simulink model "testrig_AirOilPiston_multibody"  (R2026b)
settings: Solver=daessc  StopTime=25  MaxStep=1e-2  AbsTol=1e-3
PreLoadFcn:
  | Spring = VDatabase.Spring.SUV_Landy_TA2PR_AirOilPiston_A1;
  | mass_sprung = 436.5;
  | load testrig_AirOilPiston_roughroad
undefined symbols (not defined in the file or in its folder): X, Y, Z
libraries: sm_lib x8, nesl_utility x3, fl_lib x2, Spring_AirOilPiston x1, testrig_AirOilPiston_lib x1
settings Model: Creator=Glenn  LastModifiedBy=smiller
settings SolverCC: AutoScaleAbsTol=off  MaxConsecutiveMinStep=5
settings DataIOCC: ReturnWorkspaceOutputs=off  SignalLoggingName=logsout_testrig_AirOilPiston
settings SimscapeCC: SimscapeLogLimitData=off  SimscapeLogName=simlog_testrig_AirOilPiston  SimscapeLogType=all  SimscapeUseEnergyAccounting=off
settings ExplorerConfigSet: InternalSimMechanicsExplorerSettings="<ExplorerConfiguration><canonicalview>default</canonicalview><AnimationSetting><BasePlaybackSpeed>1.0</BasePlaybackSpeed><PlaybackSpeedFactor>2.0</PlaybackSpeedFactor></AnimationSetting><TilePanel><TileInfo><Tiles Columns=\"1\" Count=\"1\" Rows=\"1\"><Column Weight=\"1\"/><Row Weight=\"1\"/><Tile Height=\"1\" Width=\"1\" X=\"0\" Y=\"0\"/></Tiles></TileInfo><SceneInfo><SceneViewer><BGColor><R>0.60000002384185791</R><G>0.60000002384185791</G><B>0.60000002384185791</B></BGColor><Camera><DoPerspective>off</DoPerspective><Position><X>0.840069872001566131</X><Y>-0.587067130109622304</Y><Z>0.736508931620452945</Z></Position><Center><X>0.0636729707701644276</X><Y>-0.0264759743902784582</Y><Z>0.448506487381626129</Z></Center><Up><X>-0.244728224943584149</X><Y>0.152949790100556315</Y><Z>0.957452065444614364</Z></Up><ViewLimDist>1</ViewLimDist><YLim>1.03004967622777266</YLim><XLim>0.912665097740277154</XLim></Camera></SceneViewer></SceneInfo></TilePanel><MechEditorPanel><Cameras/><GfxPanelCameraMap/><VideoCreator><PlaybackSpeedRatio>1.0</PlaybackSpeedRatio><FrameRate>30</FrameRate><VideoFormat>Motion JPEG AVI</VideoFormat><FrameSize>auto</FrameSize></VideoCreator></MechEditorPanel></ExplorerConfiguration>"

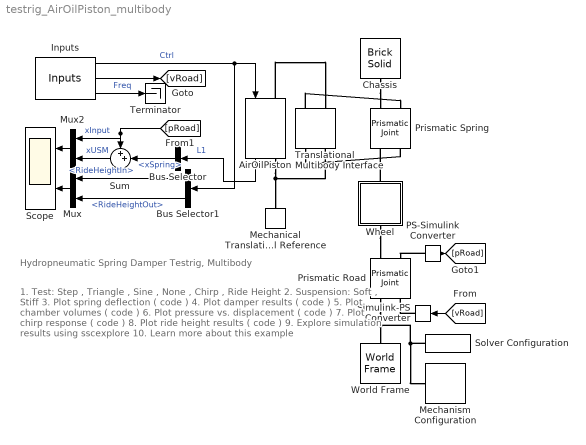
== system testrig_AirOilPiston_multibody ==
  note: 1. Test: Step , Triangle , Sine , None , Chirp , Ride Height
      | 2. Suspension: Soft , Stiff
      | 3. Plot spring deflection ( code )
      | 4. Plot damper results ( code )
      | 5. Plot chamber volumes ( code )
      | 6. Plot pressure vs. displacement ( code )
      | 7. Plot chirp response ( code )
      | 8. Plot ride height results ( code )
      | 9. Explore simulation results using sscexplore
      | 10. Learn more about this example
  note: Hydropneumatic Spring Damper Testrig, Multibody
  AirOilPiston : Spring_AirOilPiston/AirOilPiston  spr_hp_top=Spring.sTop.Value*0  spr_hp_bot=Spring.sBottom.Value*0  t_ambient=Spring.Spring.TAmbient.Value  gspr_gas_properties=Spring.Spring.GasProperties  strut_oil_properties=Spring.Strut.OilProperties  gas_chamber_soft_area=Spring.Spring.GasSoft.A.Value  gas_chamber_stiff_area=Spring.Spring.GasStiff.A.Value  gas_chamber_soft_deadvol=Spring.Spring.GasSoft.volDead.Value  gas_chamber_stiff_deadvol=Spring.Spring.GasStiff.volDead.Value  gspr_mass_soft=Spring.Spring.GasSoft.mPiston.Value  gspr_mass_stiff=Spring.Spring.GasStiff.mPiston.Value  gspr_damping_soft=Spring.Spring.GasSoft.b.Value  gspr_damping_stiff=Spring.Spring.GasStiff.b.Value  gas_chamber_soft_x0=Spring.Spring.GasSoft.xInit.Value  gas_chamber_stiff_x0=Spring.Spring.GasStiff.xInit.Value  gas_chamber_soft_p0=Spring.Spring.GasSoft.pInit.Value  gas_chamber_stiff_p0=Spring.Spring.GasStiff.pInit.Value  gspr_cwall_soft=Spring.Spring.GasSoft.CWall.Value  gspr_cwall_stiff=Spring.Spring.GasStiff.CWall.Value  oil_chamber_soft_area=Spring.Spring.OilSoft.A.Value  oil_chamber_stiff_area=Spring.Spring.OilStiff.A.Value  oil_chamber_soft_deadvol=Spring.Spring.OilSoft.volDead.Value  oil_chamber_stiff_deadvol=Spring.Spring.OilStiff.volDead.Value  oil_chamber_soft_x0=Spring.Spring.OilSoft.xInit.Value  oil_chamber_stiff_x0=Spring.Spring.OilStiff.xInit.Value  oil_chamber_soft_p0=Spring.Spring.OilSoft.pInit.Value  oil_chamber_stiff_p0=Spring.Spring.OilStiff.pInit.Value  gsprv_smax_soft=Spring.Spring.ValveSoft.xMaxOpen.Value  gsprv_smax_stiff=Spring.Spring.ValveStiff.xMaxOpen.Value  gsprv_delsmax_soft=Spring.Spring.ValveSoft.xCloseToOpen.Value  gsprv_delsmax_stiff=Spring.Spring.ValveStiff.xCloseToOpen.Value  gsprv_arealeak_soft=Spring.Spring.ValveSoft.areaLeak.Value  gsprv_arealeak_stiff=Spring.Spring.ValveStiff.areaLeak.Value  gsprv_areamax_soft=Spring.Spring.ValveSoft.aMax.Value  gsprv_areamax_stiff=Spring.Spring.ValveStiff.aMax.Value  gsprv_cd_soft=Spring.Spring.ValveSoft.Cd.Value  gsprv_cd_stiff=Spring.Spring.ValveStiff.Cd.Value  gsprv_smooth_soft=Spring.Spring.ValveSoft.smoothFactor.Value  gsprv_smooth_stiff=Spring.Spring.ValveStiff.smoothFactor.Value  gsprva_stroke_soft=Spring.Spring.ValveActuatorSoft.xStroke.Value  gsprva_stroke_stiff=Spring.Spring.ValveActuatorStiff.xStroke.Value  gsprva_ton_soft=Spring.Spring.ValveActuatorSoft.tOn.Value  gsprva_ton_stiff=Spring.Spring.ValveActuatorStiff.tOn.Value  gsprva_toff_soft=Spring.Spring.ValveActuatorSoft.tOff.Value  gsprva_toff_stiff=Spring.Spring.ValveActuatorStiff.tOff.Value  strut_deadvol=Spring.Strut.volDead.Value  strut_area=Spring.Strut.A.Value  strut_x0=Spring.Strut.xInit.Value  strut_frc_colfrc=Spring.Strut.Friction.fCoulomb.Value  strut_frc_brkfrc=Spring.Strut.Friction.fBreakaway.Value  strut_frc_brkvel=Spring.Strut.Friction.vBreakaway.Value  strut_frc_visccoeff=Spring.Strut.Friction.mu.Value  strut_p0=Spring.Strut.pInit.Value  bs_lim_upper=Spring.Endstop.xMax.Value  bs_lim_lower=Spring.Endstop.xMin.Value  bs_k_upper=Spring.Endstop.KxMax.Value  bs_k_lower=Spring.Endstop.KxMin.Value  bs_b_upper=Spring.Endstop.dxMax.Value  bs_b_lower=Spring.Endstop.dxMin.Value  bs_region=Spring.Endstop.xTransition.Value  p_diff_TLU_constant=Spring.Damper.Orifice.pDiff.Value  vol_flow_TLU_constant=Spring.Damper.Orifice.q.Value  dpr_restrarea_comp=Spring.Damper.RestrictionComp.A.Value  dpr_restrarea_reb=Spring.Damper.RestrictionReb.A.Value  dpr_cd_comp=Spring.Damper.RestrictionComp.Cd.Value  dpr_cd_reb=Spring.Damper.RestrictionReb.Cd.Value  dpr_prv_psetdiff_comp=Spring.Damper.PRVComp.pDiff.Value  dpr_prv_psetdiff_reb=Spring.Damper.PRVReb.pDiff.Value  dpr_prv_prange_comp=Spring.Damper.PRVComp.pRange.Value  dpr_prv_prange_reb=Spring.Damper.PRVReb.pRange.Value  dpr_prv_areamax_comp=Spring.Damper.PRVComp.A.Value  dpr_prv_areamax_reb=Spring.Damper.PRVReb.A.Value  dpr_prv_cd_comp=Spring.Damper.PRVComp.Cd.Value  dpr_prv_cd_reb=Spring.Damper.PRVReb.Cd.Value  dpr_cvdvalve_cmpos=Spring.CVDValve.Orifice.x.Value  dpr_cvdvalve_orifice_area=Spring.CVDValve.Orifice.A.Value  dpr_cvdvalve_orifice_pdiff=Spring.CVDValve.Orifice.pDiff.Value  dpr_cvdvalve_pcv_areamax=Spring.CVDValve.PCValve.AMax.Value  dpr_cvdvalve_pcv_prange=Spring.CVDValve.PCValve.pRange.Value  dpr_cvdvalve_arealeak=Spring.CVDValve.PCValve.ALeak.Value  dpr_cvdvalve_cd=Spring.CVDValve.PCValve.Cd.Value  dpr_cvdvalve_act_ts=Spring.CVDValve.tFilt.Value  rh_srcpressure=Spring.RideHeight.pSource.Value  rh_fcv_cmpos_inlet=Spring.RideHeight.OrificeInlet.x.Value  rh_fcv_cmpos_outlet=Spring.RideHeight.OrificeOutlet.x.Value  rh_fcv_orificearea_inlet=Spring.RideHeight.OrificeInlet.A.Value  rh_fcv_orificearea_outlet=Spring.RideHeight.OrificeOutlet.A.Value  rh_fcv_orificepdiff_inlet=Spring.RideHeight.OrificeInlet.pDiff.Value  rh_fcv_orificepdiff_outlet=Spring.RideHeight.OrificeOutlet.pDiff.Value  rh_fcv_pcprange_inlet=Spring.RideHeight.PCValveInlet.pRange.Value  rh_fcv_pcprange_outlet=Spring.RideHeight.PCValveOutlet.pRange.Value  rh_fcv_pcamax_inlet=Spring.RideHeight.PCValveInlet.AMax.Value  rh_fcv_pcamax_outlet=Spring.RideHeight.PCValveOutlet.AMax.Value  rh_fcv_arealeak_inlet=Spring.RideHeight.PCValveInlet.ALeak.Value  rh_fcv_arealeak_outlet=Spring.RideHeight.PCValveOutlet.ALeak.Value  rh_fcv_cd_inlet=Spring.RideHeight.PCValveInlet.Cd.Value  rh_fcv_cd_outlet=Spring.RideHeight.PCValveOutlet.Cd.Value  rh_fcv_smooth_inlet=Spring.RideHeight.PCValveInlet.smoothFactor.Value  rh_fcv_smooth_outlet=Spring.RideHeight.PCValveOutlet.smoothFactor.Value  rh_fcv_tfilt_inlet=Spring.RideHeight.PCValveInlet.tFilt.Value  rh_fcv_tfilt_outlet=Spring.RideHeight.PCValveOutlet.tFilt.Value
  Bus Selector : BusSelector  OutputSignals=xSpring
  Bus Selector1 : BusSelector  OutputSignals=RideHeightIn,RideHeightOut
  Chassis : sm_lib/Body Elements/Brick Solid  BrickDimensions=[1 1 0.5]  BrickDimensionsUnits=m  ExportEntireGeometry=off  InertiaType=CalculateFromGeometry  BasedOnType=Mass  Density=1000  DensityUnits=kg/m^3  Mass=mass_sprung  MassUnits=kg  CenterOfMass=[0 0 0]  CenterOfMassUnits=m  MomentsOfInertia=[1 1 1]  MomentsOfInertiaUnits=kg*m^2  ProductsOfInertia=[0 0 0]  ProductsOfInertiaUnits=kg*m^2  GraphicType=FromGeometry  MarkerShape=Sphere  MarkerSize=10  GraphicVisPropType=SimpleVisualProperties  GraphicDiffuseColor=[0.1255 0.4706 0]  GraphicOpacity=1  GraphicSpecularColor=[0.5 0.5 0.5 1.0]  GraphicAmbientColor=[0.15 0.15 0.15 1.0]  GraphicEmissiveColor=[0.0 0.0 0.0 1.0]  GraphicShininess=75  DoExposeReferenceFrame=on  SerializedFrames=<Frames/>
  Inputs : testrig_AirOilPiston_lib/Inputs  popup_suspension_stiffness=Soft  popup_rh_test_seq=None  cvd_value=1  popup_roadpz_test_type=Step  pAmp=0.05  tPer=4  nCyc=50  nCycSet=1  chirpFreqFinish=5  chirpFreqStart=0.5  chirpTimeFinish=20  chirpTimeStart=5  spdkmh=10  roughTimeStart=5
      settings: AttributesFormatString=|
      | Road Height: %<popup_roadpz_test_type>
      | Suspension: %<popup_suspension_stiffness>
      | Ride Height: %<popup_rh_test_seq>
  Mechanical Translational Reference : fl_lib/Mechanical/Translational Elements/Mechanical Translational Reference
  Mechanism Configuration : sm_lib/Utilities/Mechanism Configuration  UniformGravity=Constant  GravityVector=[0 0 -9.80665]  GravityVectorUnits=m/s^2  LinearizationDelta=0.001  JointModeTransitionNonlinearIterations=2
  Mux : Mux  Inputs=2
  Mux2 : Mux  Inputs=2
  PS-Simulink Converter : nesl_utility/PS-Simulink Converter  PhysicalDomain=network_engine_domain  SubClassName=ps_output  LeftPortType=input  RightPortType=output  PseudoPeriodic=off  Frequencies=[]  VectorFormat=inherit  Unit=inherit  AffineConversion=off
  Prismatic Road : sm_lib/Joints/Prismatic Joint  JointMode=Normal  CompositeWrenchDir=FollowerOnBase  CompositeWrenchFrame=BaseFrame  SenseConstraintForce=off  SenseConstraintTorque=off  SenseTotalForce=off  SenseTotalTorque=off  PositionTargetSpecify=off  PositionTargetPriority=High  PositionTargetValue=0  PositionTargetValueUnits=m  VelocityTargetSpecify=off  VelocityTargetPriority=High  VelocityTargetValue=0  VelocityTargetValueUnits=m/s  EquilibriumPosition=0  EquilibriumPositionUnits=m  SpringStiffness=0  SpringStiffnessUnits=N/m  DampingCoefficient=0  DampingCoefficientUnits=N/(m/s)  LowerLimitSpecify=off  LowerLimitBound=-1  LowerLimitBoundUnits=m  LowerLimitStiffness=1e6  LowerLimitStiffnessUnits=N/m  LowerLimitDamping=1e3  LowerLimitDampingUnits=N/(m/s)  LowerLimitTransitionRegionWidth=1e-4  LowerLimitTransitionRegionWidthUnits=m  UpperLimitSpecify=off  UpperLimitBound=1  UpperLimitBoundUnits=m  UpperLimitStiffness=1e6  UpperLimitStiffnessUnits=N/m  UpperLimitDamping=1e3  UpperLimitDampingUnits=N/(m/s)  UpperLimitTransitionRegionWidth=1e-4  UpperLimitTransitionRegionWidthUnits=m  TorqueActuationMode=ComputedTorque  MotionActuationMode=InputMotion  SensePosition=on  SenseVelocity=off  SenseAcceleration=off  SenseTorqueForce=off  SenseLowerLimitTorqueForce=off  SenseUpperLimitTorqueForce=off
  Prismatic Spring : sm_lib/Joints/Prismatic Joint  JointMode=Normal  CompositeWrenchDir=FollowerOnBase  CompositeWrenchFrame=BaseFrame  SenseConstraintForce=off  SenseConstraintTorque=off  SenseTotalForce=off  SenseTotalTorque=off  PositionTargetSpecify=off  PositionTargetPriority=High  PositionTargetValue=0  PositionTargetValueUnits=m  VelocityTargetSpecify=off  VelocityTargetPriority=High  VelocityTargetValue=0  VelocityTargetValueUnits=m/s  EquilibriumPosition=0  EquilibriumPositionUnits=m  SpringStiffness=0  SpringStiffnessUnits=N/m  DampingCoefficient=0  DampingCoefficientUnits=N/(m/s)  LowerLimitSpecify=off  LowerLimitBound=-1  LowerLimitBoundUnits=m  LowerLimitStiffness=1e6  LowerLimitStiffnessUnits=N/m  LowerLimitDamping=1e3  LowerLimitDampingUnits=N/(m/s)  LowerLimitTransitionRegionWidth=1e-4  LowerLimitTransitionRegionWidthUnits=m  UpperLimitSpecify=off  UpperLimitBound=1  UpperLimitBoundUnits=m  UpperLimitStiffness=1e6  UpperLimitStiffnessUnits=N/m  UpperLimitDamping=1e3  UpperLimitDampingUnits=N/(m/s)  UpperLimitTransitionRegionWidth=1e-4  UpperLimitTransitionRegionWidthUnits=m  TorqueActuationMode=InputTorque  MotionActuationMode=ComputedMotion  SensePosition=off  SenseVelocity=on  SenseAcceleration=off  SenseTorqueForce=off  SenseLowerLimitTorqueForce=off  SenseUpperLimitTorqueForce=off
  Scope : Scope  NumInputPorts=2
      settings: ActiveDisplayYMinimum=-0.12106  ActiveDisplayYMaximum=0.26576
  Simulink-PS Converter : nesl_utility/Simulink-PS Converter  PhysicalDomain=network_engine_domain  SubClassName=ps_input  LeftPortType=input  RightPortType=output  PseudoPeriodic=off  Frequencies=[]  NoiseDistribution=none  NoiseParameters=[]  Unit=m  AffineConversion=off  FilteringAndDerivatives=filter  SimscapeFilterOrder=2  InputFilterTimeConstant=0.001  UdotUserProvided=0
  Solver Configuration : nesl_utility/Solver Configuration  PhysicalDomain=network_engine_domain  SubClassName=solver  LeftPortType=input  RightPortType=generic  Tones=[]  Harmonics=[]  SimulateNoise=off  Profile=off  UseLocalSampling=off  EnableSwitchedLinearOptims=on  FrequencyDomain=off  UseCCode=off  RelTol=0.001  AbsTol=0.001  MinStep=1e-09  ToWorkspace=off  RevertToSquareIcSolve=off  NumHomotopyIterations=100  PhasorMode=off  PhasorModeNumHarmonics=1  ConsistencySolver=NEWTON_FTOL  CanonicalOrdering=UNORDERED  OptimizeIntermediates=UNOPTIMIZED  MulticoreSolverChoice=BACKWARD_EULER  IndexReductionMethod=DerivativeReplacement  DoDC=off  ResidualTolerance=1e-09  ConsistencyTolSource=GLOBAL  ConsistencyAbsTol=0.001  ConsistencyRelTol=0.001  ConsistencyTolFactor=0.001  UseLocalSolver=off  LocalSolverChoice=NE_BACKWARD_EULER_ADVANCER  ResolveIndetEquations=on  FunctionEvalNumThread=1  LocalSolverSampleTime=0.001  DoFixedCost=off  MaxNonlinIter=3  MaxModeIter=2  ComputeImpulses=off  ImpulseIterations=2  LinearAlgebra=auto  LinearAlgebraNumThread=0  EquationFormulation=NE_TIME_EF  DelaysMemoryBudget=1024  AutomaticFiltering=on  FilteringTimeConstant=0.001  PartitionStorageMethod=AS_NEEDED  PartitionMemoryBudget=1024  PartitionMethod=BALANCED  MultibodyUseLocalSolver=off  MultibodyLocalSolverChoice=ODE1  MultibodyLocalSolverSampleTime=0.001
  Sum : Sum  Inputs=++|
  Terminator : Terminator
  Translational Multibody Interface : fl_lib/Mechanical/Multibody Interfaces/Translational Multibody Interface
  Wheel : Subsystem
  World Frame : sm_lib/Frames and Transforms/World Frame
  wires:
  AirOilPiston/1 -> Bus Selector/1  "L1"
  Sum/1 -> Mux2/2  "xUSM"
  Mux/1 -> Scope/2
  Bus Selector1/1 -> Mux/1  "<RideHeightIn>"
  Bus Selector1/2 -> Mux/2  "<RideHeightOut>"
  Inputs/1 -> Bus Selector1/1, AirOilPiston/1  "Ctrl"
  Mux2/1 -> Scope/1
  PS-Simulink Converter/1 -> [pRoad]
  [vRoad] -> Simulink-PS Converter/1
  [pRoad] -> Mux2/1, Sum/1  "xInput"
  Inputs/2 -> [vRoad]
  Bus Selector/1 -> Sum/2  "<xSpring>"
  Inputs/3 -> Terminator/1  "Freq"
  connections:
  AirOilPiston/RConn1 -- Translational Multibody Interface/LConn2 -- Mechanical Translational Reference/LConn1
  AirOilPiston/LConn1 -- Translational Multibody Interface/RConn2
  Translational Multibody Interface/LConn1 -- Prismatic Spring/LConn2
  Translational Multibody Interface/RConn1 -- Prismatic Spring/RConn2
  Chassis/RConn1 -- Prismatic Spring/RConn1
  Prismatic Road/LConn1 -- Mechanism Configuration/RConn1 -- Solver Configuration/RConn1 -- World Frame/RConn1
  Simulink-PS Converter/RConn1 -- Prismatic Road/LConn2
  PS-Simulink Converter/LConn1 -- Prismatic Road/RConn2
  Wheel/LConn1 -- Prismatic Spring/LConn1
  Wheel/RConn1 -- Prismatic Road/RConn1

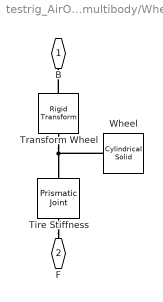
== system testrig_AirOilPiston_multibody/Wheel ==
  Tire Stiffness : sm_lib/Joints/Prismatic Joint  JointMode=Normal  CompositeWrenchDir=FollowerOnBase  CompositeWrenchFrame=BaseFrame  SenseConstraintForce=off  SenseConstraintTorque=off  SenseTotalForce=off  SenseTotalTorque=off  PositionTargetSpecify=off  PositionTargetPriority=High  PositionTargetValue=0  PositionTargetValueUnits=m  VelocityTargetSpecify=off  VelocityTargetPriority=High  VelocityTargetValue=0  VelocityTargetValueUnits=m/s  EquilibriumPosition=0  EquilibriumPositionUnits=m  SpringStiffness=3.9759e+05  SpringStiffnessUnits=N/m  DampingCoefficient=3.9759e+05*0.1  DampingCoefficientUnits=N/(m/s)  LowerLimitSpecify=off  LowerLimitBound=-1  LowerLimitBoundUnits=m  LowerLimitStiffness=1e6  LowerLimitStiffnessUnits=N/m  LowerLimitDamping=1e3  LowerLimitDampingUnits=N/(m/s)  LowerLimitTransitionRegionWidth=1e-4  LowerLimitTransitionRegionWidthUnits=m  UpperLimitSpecify=off  UpperLimitBound=1  UpperLimitBoundUnits=m  UpperLimitStiffness=1e6  UpperLimitStiffnessUnits=N/m  UpperLimitDamping=1e3  UpperLimitDampingUnits=N/(m/s)  UpperLimitTransitionRegionWidth=1e-4  UpperLimitTransitionRegionWidthUnits=m  TorqueActuationMode=NoTorque  MotionActuationMode=ComputedMotion  SensePosition=off  SenseVelocity=off  SenseAcceleration=off  SenseTorqueForce=off  SenseLowerLimitTorqueForce=off  SenseUpperLimitTorqueForce=off
  Transform Wheel : sm_lib/Frames and Transforms/Rigid Transform  RotationMethod=None  FollAlignAxisA=+X  BaseAlignAxisA=+Y  FollAlignAxisB=+Y  BaseAlignAxisB=+Z  RotationStandardAxis=+Z  RotationAngle=0  RotationAngleUnits=deg  RotationArbitraryAxis=[0 0 1]  RotationSequenceAxes=FollowerAxes  RotationSequence=XYX  RotationSequenceAngles=[0 0 0]  RotationSequenceAnglesUnits=deg  RotationMatrix=[1 0 0;0 1 0;0 0 1]  Quaternion=[1 0 0 0]  TranslationMethod=StandardAxis  TranslationCartesianOffset=[0 0 0]  TranslationCartesianOffsetUnits=m  TranslationStandardAxis=+Z  TranslationStandardOffset=-0.5  TranslationStandardOffsetUnits=m  TranslationROffset=0  TranslationROffsetUnits=m  TranslationThetaOffset=0  TranslationThetaOffsetUnits=deg  TranslationZOffset=0  TranslationZOffsetUnits=m
  Wheel : sm_lib/Body Elements/Cylindrical Solid  CylinderRadius=0.35  CylinderRadiusUnits=m  CylinderLength=0.1  CylinderLengthUnits=m  ExportEntireGeometry=off  InertiaType=CalculateFromGeometry  BasedOnType=Density  Density=1000  DensityUnits=kg/m^3  Mass=1  MassUnits=kg  CenterOfMass=[0 0 0]  CenterOfMassUnits=m  MomentsOfInertia=[1 1 1]  MomentsOfInertiaUnits=kg*m^2  ProductsOfInertia=[0 0 0]  ProductsOfInertiaUnits=kg*m^2  GraphicType=FromGeometry  MarkerShape=Sphere  MarkerSize=10  GraphicVisPropType=SimpleVisualProperties  GraphicDiffuseColor=[0.5 0.5 0.5]  GraphicOpacity=1  GraphicSpecularColor=[0.5 0.5 0.5 1.0]  GraphicAmbientColor=[0.15 0.15 0.15 1.0]  GraphicEmissiveColor=[0.0 0.0 0.0 1.0]  GraphicShininess=75  DoExposeReferenceFrame=off  SerializedFrames=<Frames><Frame><Id>Frame1</Id><Value><Name>F1</Name><Origin><Source>ReferenceFrame</Source><FeatureName></FeatureName></Origin><PrimaryAxis><DefinedDirection>+X</DefinedDirection><Source>ReferenceFrame</Source><SourceDirection>+Z</SourceDirection><FeatureName></FeatureName></PrimaryAxis><SecondaryAxis><DefinedDirection>+Y</DefinedDirection><Source>ReferenceFrame</Source><SourceDirection>+Y</SourceDirection><FeatureName></FeatureName></SecondaryAxis></Value></Frame></Frames>
  B : PMIOPort  Side=Left
  F : PMIOPort  Port=2  Side=Right
  connections:
  Transform Wheel/RConn1 -- Wheel/LConn1 -- Tire Stiffness/RConn1
  Transform Wheel/LConn1 -- B/RConn1
  Tire Stiffness/LConn1 -- F/RConn1
